simulink model "lfp_pack_plant"  (R2025a)
settings: Solver=daessc  StartTime=0.0  StopTime=t_stop  MaxStep=1  RelTol=1e-3
undefined symbols (not defined in the file): bal_dV, bal_enable, bal_Ts, SOC_stop, T_amb_K
libraries: fl_lib x7, nesl_utility x6, lfp_pack16s_lib x1, simulink x1
settings Model: Creator=hari2  LastModifiedBy=hari2
settings DataIOCC: SaveOutput=off  SaveTime=off

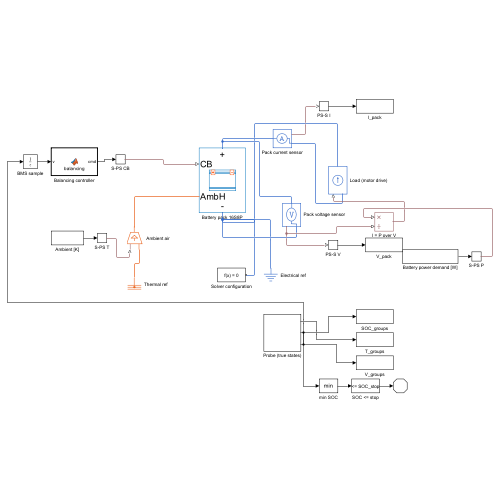
[thumbnail: Simulink's stored preview of the top-level diagram]
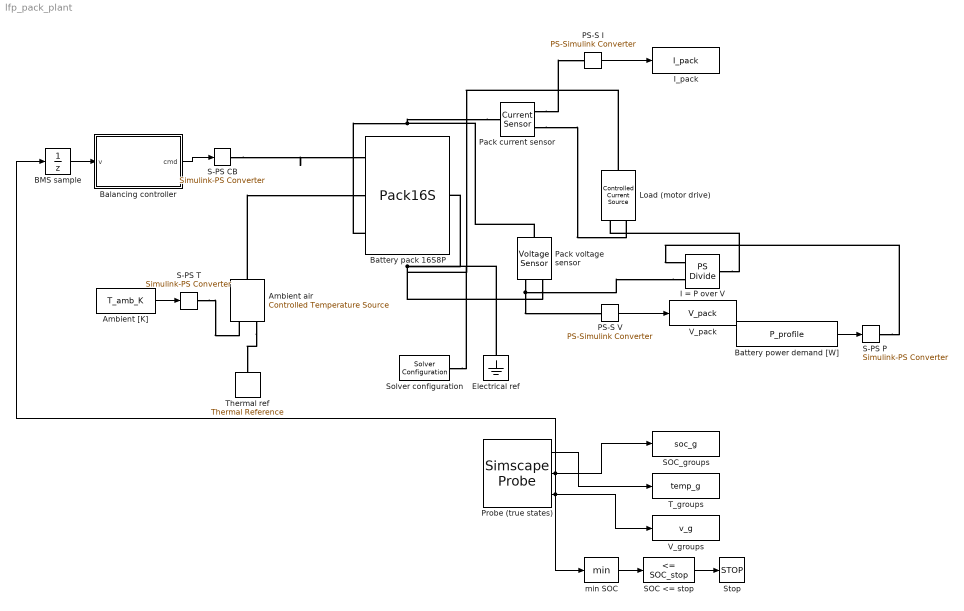
== system lfp_pack_plant ==
  Ambient [K] : Constant  Value=T_amb_K
  Ambient air : fl_lib/Thermal/Thermal Sources/Controlled Temperature Source
  BMS sample : UnitDelay  InitialCondition=3.3*ones(16,1)  SampleTime=bal_Ts  HasFrameUpgradeWarning=on
  Balancing controller : MATLAB Function  TreatAsAtomicUnit=on
  Battery pack 16S8P : lfp_pack16s_lib/Pack16S  BatteryCapacityCell=Pack16S.BatteryCapacityCell A*hr  BatteryCapacityCellPercentDeviation=Pack16S.BatteryCapacityCellPercentDeviation  ExtrapolationMethodCell=simscape.enum.extrapolation.nearest  SOCBreakpointsCell=Pack16S.SOCBreakpointsCell  SOCBreakpointsCellPercentDeviation=Pack16S.SOCBreakpointsCellPercentDeviation  TemperatureBreakpointsCell=Pack16S.TemperatureBreakpointsCell K  TemperatureBreakpointsCellPercentDeviation=Pack16S.TemperatureBreakpointsCellPercentDeviation  OpenCircuitVoltageThermalCell=Pack16S.OpenCircuitVoltageThermalCell V  OpenCircuitVoltageThermalCellPercentDeviation=Pack16S.OpenCircuitVoltageThermalCellPercentDeviation  VoltageRangeCell=Pack16S.VoltageRangeCell V  VoltageRangeCellPercentDeviation=Pack16S.VoltageRangeCellPercentDeviation  MaximumHysteresisVoltageThermalCell=Pack16S.MaximumHysteresisVoltageThermalCell V  MaximumHysteresisVoltageThermalCellPercentDeviation=Pack16S.MaximumHysteresisVoltageThermalCellPercentDeviation  InstantaneousHysteresisVoltageThermalCell=Pack16S.InstantaneousHysteresisVoltageThermalCell V  InstantaneousHysteresisVoltageThermalCellPercentDeviation=Pack16S.InstantaneousHysteresisVoltageThermalCellPercentDeviation  HysteresisRateThermalCell=Pack16S.HysteresisRateThermalCell  HysteresisRateThermalCellPercentDeviation=Pack16S.HysteresisRateThermalCellPercentDeviation  ResistanceSOCBreakpointsCell=Pack16S.ResistanceSOCBreakpointsCell  ResistanceSOCBreakpointsCellPercentDeviation=Pack16S.ResistanceSOCBreakpointsCellPercentDeviation  ResistanceTemperatureBreakpointsCell=Pack16S.ResistanceTemperatureBreakpointsCell K  ResistanceTemperatureBreakpointsCellPercentDeviation=Pack16S.ResistanceTemperatureBreakpointsCellPercentDeviation  R0ThermalCell=Pack16S.R0ThermalCell Ohm  R0ThermalCellPercentDeviation=Pack16S.R0ThermalCellPercentDeviation  R1ThermalCell=Pack16S.R1ThermalCell Ohm  R1ThermalCellPercentDeviation=Pack16S.R1ThermalCellPercentDeviation  Tau1ThermalCell=Pack16S.Tau1ThermalCell s  Tau1ThermalCellPercentDeviation=Pack16S.Tau1ThermalCellPercentDeviation  R2ThermalCell=Pack16S.R2ThermalCell Ohm  R2ThermalCellPercentDeviation=Pack16S.R2ThermalCellPercentDeviation  Tau2ThermalCell=Pack16S.Tau2ThermalCell s  Tau2ThermalCellPercentDeviation=Pack16S.Tau2ThermalCellPercentDeviation  BatteryThermalMassCell=Pack16S.BatteryThermalMassCell J/K  BatteryThermalMassCellPercentDeviation=Pack16S.BatteryThermalMassCellPercentDeviation  AmbientResistance=Pack16S.AmbientResistance K/W  InterParallelAssemblyThermalResistance=Pack16S.InterParallelAssemblyThermalResistance K/W  CellBalancingClosedResistance=Pack16S.CellBalancingClosedResistance Ohm  CellBalancingOpenConductance=Pack16S.CellBalancingOpenConductance 1/Ohm  CellBalancingThreshold=Pack16S.CellBalancingThreshold  CellBalancingResistance=Pack16S.CellBalancingResistance Ohm  P=8  S=16  NumInterParallelAssemblyThermalConnections=15  InterParallelAssemblyConnectionsMapping=[1, 2, 3, 4, 5, 6, 7, 8, 9, 10, 11, 12, 13, 14, 15; 2, 3, 4, 5, 6, 7, 8, 9, 10, 11, 12, 13, 14, 15, 16]  InterParallelAssemblyConnectionParameterScaleUp=[1, 1, 1, 1, 1, 1, 1, 1, 1, 1, 1, 1, 1, 1, 1]  SeriesGrouping=[1, 1, 1, 1, 1, 1, 1, 1, 1, 1, 1, 1, 1, 1, 1, 1]  ParallelGrouping=[1, 1, 1, 1, 1, 1, 1, 1, 1, 1, 1, 1, 1, 1, 1, 1]  socCell_specify=on  socCell_priority=High  socCell=SOC0_vec  socCell_nominal_specify=off  socCell_nominal_value=1  socCell_nominal_unit=1  batteryVoltage_specify=off  batteryVoltage_priority=None  batteryVoltage=repmat(0, 16, 1) V  batteryVoltage_nominal_specify=off  batteryVoltage_nominal_value=1  batteryVoltage_nominal_unit=V  batteryCurrent_specify=off  batteryCurrent_priority=None  batteryCurrent=repmat(0, 16, 1) A  batteryCurrent_nominal_specify=off  batteryCurrent_nominal_value=1  batteryCurrent_nominal_unit=A  numCycles_specify=off  numCycles_priority=High  numCycles=repmat(0, 16, 1)  numCycles_nominal_specify=off  numCycles_nominal_value=1  numCycles_nominal_unit=1  batteryTemperature_specify=on  batteryTemperature_priority=High  batteryTemperature=T0_vec_K K  batteryTemperature_nominal_specify=off  batteryTemperature_nominal_value=1  batteryTemperature_nominal_unit=K  hysteresisState_specify=on  hysteresisState_priority=High  hysteresisState=h0_vec  hysteresisState_nominal_specify=off  hysteresisState_nominal_value=1  hysteresisState_nominal_unit=1  vParallelAssembly_specify=off  vParallelAssembly_priority=None  vParallelAssembly=repmat(0, 16, 1) V  vParallelAssembly_nominal_specify=off  vParallelAssembly_nominal_value=1  vParallelAssembly_nominal_unit=V  socParallelAssembly_specify=off  socParallelAssembly_priority=None  socParallelAssembly=repmat(1, 16, 1)  socParallelAssembly_nominal_specify=off  socParallelAssembly_nominal_value=1  socParallelAssembly_nominal_unit=1
      settings: InternalSimscapePortConfiguration="{\"Bottom\":[{\"id\":\"n\",\"label\":\"-\",\"type\":\"foundation.electrical.electrical\"}],\"Left\":[{\"id\":\"enableCellBalancing\",\"label\":\"CB\",\"type\":\"input\"},{\"id\":\"AmbH\",\"label\":\"AmbH\",\"type\":\"foundation.thermal.thermal\"}],\"Right\":[],\"Top\":[{\"id\":\"p\",\"label\":\"+\",\"type\":\"foundation.electrical.electrical\"}]}"
  Battery power demand [W] : FromWorkspace  VariableName=P_profile  Interpolate=off  OutputAfterFinalValue=Holding final value
  Electrical ref : fl_lib/Electrical/Electrical Elements/Electrical Reference
  I = P over V : fl_lib/Physical Signals/Functions/PS Divide
  I_pack : ToWorkspace  VariableName=I_pack  SampleTime=[1 0.5]
  Load (motor drive) : fl_lib/Electrical/Electrical Sources/Controlled Current Source
  PS-S I : nesl_utility/PS-Simulink Converter  PhysicalDomain=network_engine_domain  SubClassName=ps_output  LeftPortType=input  RightPortType=output  PseudoPeriodic=off  Frequencies=[]  VectorFormat=inherit  Unit=A  AffineConversion=off
  PS-S V : nesl_utility/PS-Simulink Converter  PhysicalDomain=network_engine_domain  SubClassName=ps_output  LeftPortType=input  RightPortType=output  PseudoPeriodic=off  Frequencies=[]  VectorFormat=inherit  Unit=V  AffineConversion=off
  Pack current sensor : fl_lib/Electrical/Electrical Sensors/Current Sensor
  Pack voltage sensor : fl_lib/Electrical/Electrical Sensors/Voltage Sensor
  Probe (true states) : SimscapeProbe  BoundBlock=1  Variables="{\"batteryTemperature\":{\"Probing\":\"ON\"},\"socCell\":{\"Probing\":\"ON\"},\"vParallelAssembly\":{\"Probing\":\"ON\"}}"
  S-PS CB : nesl_utility/Simulink-PS Converter  PhysicalDomain=network_engine_domain  SubClassName=ps_input  LeftPortType=input  RightPortType=output  PseudoPeriodic=off  Frequencies=[]  NoiseDistribution=none  NoiseParameters=[]  Unit=1  AffineConversion=off  FilteringAndDerivatives=provide  SimscapeFilterOrder=1  InputFilterTimeConstant=0.001  UdotUserProvided=0
  S-PS P : nesl_utility/Simulink-PS Converter  PhysicalDomain=network_engine_domain  SubClassName=ps_input  LeftPortType=input  RightPortType=output  PseudoPeriodic=off  Frequencies=[]  NoiseDistribution=none  NoiseParameters=[]  Unit=W  AffineConversion=off  FilteringAndDerivatives=filter  SimscapeFilterOrder=1  InputFilterTimeConstant=0.1  UdotUserProvided=0
  S-PS T : nesl_utility/Simulink-PS Converter  PhysicalDomain=network_engine_domain  SubClassName=ps_input  LeftPortType=input  RightPortType=output  PseudoPeriodic=off  Frequencies=[]  NoiseDistribution=none  NoiseParameters=[]  Unit=K  AffineConversion=off  FilteringAndDerivatives=provide  SimscapeFilterOrder=1  InputFilterTimeConstant=0.001  UdotUserProvided=0
  SOC <= stop : simulink/Logic and Bit Operations/Compare To Constant  relop=<=  const=SOC_stop  OutDataTypeStr=boolean
  SOC_groups : ToWorkspace  VariableName=soc_g  SampleTime=[1 0.5]
  Solver configuration : nesl_utility/Solver Configuration  PhysicalDomain=network_engine_domain  SubClassName=solver  LeftPortType=input  RightPortType=generic  Tones=[]  Harmonics=[]  SimulateNoise=off  Profile=off  UseLocalSampling=off  EnableSwitchedLinearOptims=on  FrequencyDomain=off  UseCCode=off  RelTol=0.001  AbsTol=0.001  MinStep=1e-09  ToWorkspace=off  RevertToSquareIcSolve=off  NumHomotopyIterations=100  PhasorMode=off  PhasorModeNumHarmonics=1  ConsistencySolver=NEWTON_XTOL_AFTER_FTOL  IndexReductionMethod=DerivativeReplacement  DoDC=off  ResidualTolerance=1e-09  ConsistencyTolSource=GLOBAL  ConsistencyAbsTol=0.001  ConsistencyRelTol=0.001  ConsistencyTolFactor=0.001  UseLocalSolver=off  LocalSolverChoice=NE_BACKWARD_EULER_ADVANCER  ResolveIndetEquations=on  FunctionEvalNumThread=1  LocalSolverSampleTime=0.001  DoFixedCost=off  MaxNonlinIter=3  MaxModeIter=2  ComputeImpulses=off  ImpulseIterations=2  LinearAlgebra=auto  LinearAlgebraNumThread=0  EquationFormulation=NE_TIME_EF  DelaysMemoryBudget=1024  AutomaticFiltering=on  FilteringTimeConstant=0.001  PartitionStorageMethod=AS_NEEDED  PartitionMemoryBudget=1024  PartitionMethod=ROBUST  MultibodyUseLocalSolver=off  MultibodyLocalSolverChoice=ODE1  MultibodyLocalSolverSampleTime=0.001
  Stop : Stop
  T_groups : ToWorkspace  VariableName=temp_g  SampleTime=[1 0.5]
  Thermal ref : fl_lib/Thermal/Thermal Elements/Thermal Reference
  V_groups : ToWorkspace  VariableName=v_g  SampleTime=[1 0.5]
  V_pack : ToWorkspace  VariableName=V_pack  SampleTime=[1 0.5]
  min SOC : MinMax
  wires:
  Battery power demand [W]/1 -> S-PS P/1
  Ambient [K]/1 -> S-PS T/1
  Balancing controller/1(cmd) -> S-PS CB/1
  PS-S I/1 -> I_pack/1
  PS-S V/1 -> V_pack/1
  Probe (true states)/2 -> SOC_groups/1, min SOC/1
  Probe (true states)/1 -> T_groups/1
  Probe (true states)/3 -> V_groups/1, BMS sample/1
  BMS sample/1 -> Balancing controller/1(v)
  min SOC/1 -> SOC <= stop/1
  SOC <= stop/1 -> Stop/1
  connections:
  Pack current sensor/LConn1 -- Battery pack 16S8P/LConn3 -- Pack voltage sensor/LConn1
  Pack current sensor/RConn2 -- Load (motor drive)/RConn2
  Load (motor drive)/LConn1 -- Pack voltage sensor/RConn2 -- Electrical ref/LConn1 -- Battery pack 16S8P/RConn1 -- Solver configuration/RConn1
  Ambient air/LConn1 -- Battery pack 16S8P/LConn2
  Ambient air/RConn2 -- Thermal ref/LConn1
  S-PS P/RConn1 -- I = P over V/LConn1
  I = P over V/LConn2 -- Pack voltage sensor/RConn1 -- PS-S V/LConn1
  I = P over V/RConn1 -- Load (motor drive)/RConn1
  S-PS T/RConn1 -- Ambient air/RConn1
  S-PS CB/RConn1 -- Battery pack 16S8P/LConn1
  Pack current sensor/RConn1 -- PS-S I/LConn1

== matlab function lfp_pack_plant/Balancing controller ==
  data: v input size=[16 1]; cmd output size=[16 1]; bal_enable parameter; bal_dV parameter
function cmd = balancing(v, bal_enable, bal_dV)
% Voltage-based passive balancing, as in typical 2W BMS chips.
% v: group voltages [V]; bal_enable: 1 = balancing allowed; bal_dV: threshold [V]
cmd = zeros(size(v));
if bal_enable > 0.5
    cmd = double(v > min(v) + bal_dV);
end
